simulink model "pendulum_pid"  (R2025b)
settings: Solver=ode45  StartTime=0.0  StopTime=8  MaxStep=1e-3  RelTol=1e-6
values from neighbouring files (symbols this model uses):
  A = reshape(p(1:16),4,4)    [main_pid_inverted_pendulum.m]    (also in params.m = [0  1         0                  0)
  B = p(17:20)'; [Kp,Ki,Kd,N] = deal(p(21),p(22),p(23),p(24))    [main_pid_inverted_pendulum.m]    (also in params.m = [0; J/D; 0; -m*l/D])
  Cfull = eye(4)    [compare_pid_vs_assy.m]
  Dfull = zeros(4,1)    [build_simulink_pid_model.m]    (also in compare_pid_vs_assy.m)
  Kd = -645.6    [main_pid_inverted_pendulum.m]    (also in optimize_pid.m = K(3); pid_gains.mat)
  Ki = -8365.6    [main_pid_inverted_pendulum.m]    (also in optimize_pid.m = K(2); pid_gains.mat)
  Kp = -4192.9    [main_pid_inverted_pendulum.m]    (also in optimize_pid.m = K(1); pid_gains.mat)
  Tf = 1/100    (= 0.01)    [main_pid_inverted_pendulum.m]    (also in optimize_pid.m; pid_gains.mat)
  th0 = asin(0.023848750116849705)    [params.m]
  x0 = [0; 0; th0; 0]    [build_simulink_pid_model.m]    (also in compare_pid_vs_assy.m; optimize_pid.m = [0;0;1;0;0;-1])
libraries: slpidlib x1
settings Model: Creator=kSam  LastModifiedBy=kSam

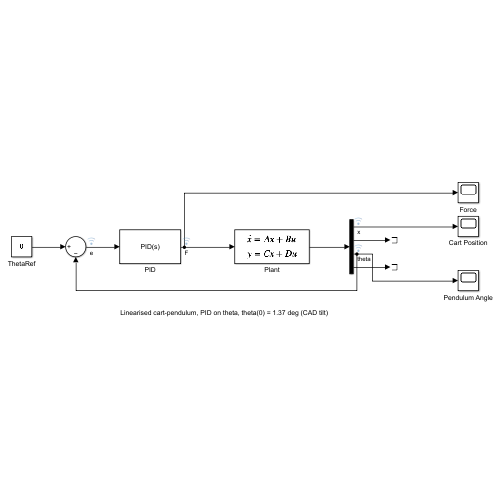
[thumbnail: Simulink's stored preview of the top-level diagram]
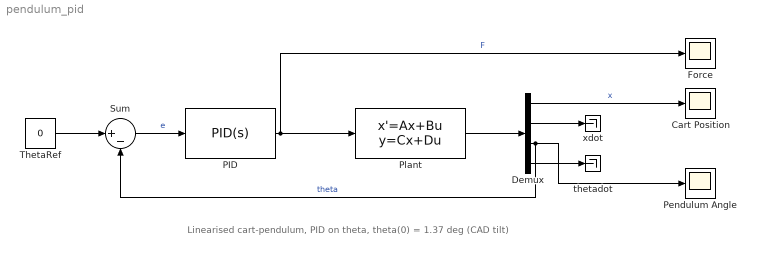
== system pendulum_pid ==
  note: Linearised cart-pendulum, PID on theta, theta(0) = 1.37 deg (CAD tilt)
  Cart Position : Scope
      settings: TimeSpan=8  Title=Cart position x  ActiveDisplayYMinimum=-0.005  ActiveDisplayYMaximum=0.035  YLabel=x [m]
  Demux : Demux
  Force : Scope
      settings: TimeSpan=8  Title=Control force F  ActiveDisplayYMinimum=-20  ActiveDisplayYMaximum=110  YLabel=F [N]
  PID : slpidlib/PID Controller  Controller=PID  Form=Parallel  TimeDomain=Continuous-time  UseExternalTs=off  SampleTime=-1  IntegratorMethod=Forward Euler  FilterMethod=Forward Euler  ControllerParametersSource=internal  P=Kp  I=Ki  UseKiTs=off  D=Kd  UseExternalDerivativeSource=off  N=1/Tf  UseFilter=on  TunerSelectOption=Transfer Function Based (PID Tuner App)  InitialConditionSource=internal  InitialConditionForIntegrator=0  InitialConditionForFilter=Kd*(-th0)  DifferentiatorICPrevScaledInput=0  ExternalReset=none  TrackingMode=off  Kt=1  LimitOutput=off  SatLimitsSource=internal  UpperSaturationLimit=inf  LowerSaturationLimit=-inf  LinearizeAsGain=on  AntiWindupMode=none  Kb=1  LimitIntegrator=off  UpperIntegratorSaturationLimit=inf  LowerIntegratorSaturationLimit=-inf  POutMin=[]  POutMax=[]  IOutMin=[]  IOutMax=[]  DOutMin=[]  DOutMax=[]  NOutMin=[]  NOutMax=[]  SumOutMin=[]  SumOutMax=[]  SaturationOutMin=[]  SaturationOutMax=[]  PParamMin=[]  PParamMax=[]  IParamMin=[]  IParamMax=[]  DParamMin=[]  DParamMax=[]  NParamMin=[]  NParamMax=[]  KbParamMin=[]  KbParamMax=[]  KtParamMin=[]  KtParamMax=[]  KbOutMin=[]  KbOutMax=[]  KtOutMin=[]  KtOutMax=[]  IntegratorOutMin=[]  IntegratorOutMax=[]  FilterOutMin=[]  FilterOutMax=[]  SumI1OutMin=[]  SumI1OutMax=[]  SumI2OutMin=[]  SumI2OutMax=[]  SumI3OutMin=[]  SumI3OutMax=[]  SumI4OutMin=[]  SumI4OutMax=[]  SumDOutMin=[]  SumDOutMax=[]  DifferentiatorOutMin=[]  DifferentiatorOutMax=[]  FilterDiffOutCoefMin=[]  FilterDiffOutCoefMax=[]  ReciprocalOutMin=[]  ReciprocalOutMax=[]  SumDenOutMin=[]  SumDenOutMax=[]  SumNumOutMin=[]  SumNumOutMax=[]  DivideOutMin=[]  DivideOutMax=[]  UdiffTsProdOutMin=[]  UdiffTsProdOutMax=[]  NTsProdOutMin=[]  NTsProdOutMax=[]  UintegralTsProdOutMin=[]  UintegralTsProdOutMax=[]  UngainTsProdOutMin=[]  UngainTsProdOutMax=[]  ClampingZeroOutDataTypeStr=Inherit: Inherit via back propagation  ClampingZeroOutMin=[]  ClampingZeroOutMax=[]  FilterDenConstantOutDataTypeStr=Inherit: Inherit via back propagation  FilterDenConstantOutMin=[]  FilterDenConstantOutMax=[]  PCopyOutDataTypeStr=Inherit: Inherit via back propagation  PCopyOutMin=[]  PCopyOutMax=[]  NCopyOutDataTypeStr=Inherit: Inherit via back propagation  NCopyOutMin=[]  NCopyOutMax=[]  IntegratorContinuousStateAttributes=''  IntegratorStateMustResolveToSignalObject=off  IntegratorRTWStateStorageClass=Auto  FilterContinuousStateAttributes=''  FilterStateMustResolveToSignalObject=off  FilterRTWStateStorageClass=Auto  ParallelPVariant=InternalParameters  IdealPVariant=Disabled  IVariant=InternalParameters  DVariant=InternalParameters  IntegratorVariant=Continuous  SatVariant=Disabled  AWVariant=Passthrough  PCopyVariant=Disabled  TRVariant=Disabled  FdbkBlocksVariant=Forward  IdealPFdbkVariant=Disabled  SatFdbkVariant=Disabled  DerivativeFilterVariant=ContFilter  NVariant=InternalParameters  NCopyVariant=Disabled  FilterICVariant=InternalICsFilter  IntegratorICVariant=InternalICs  ExternalResetVariant=Disabled  TRSumVariant=Passthrough  SumFdbkVariant=Disabled  SumVariant=Sum_PID  TsampFilterVariant=InternalTs  TsampNgainVariant=Passthrough  TsampIntegralVariant=Disabled_SignalSpec  ExternalSaturationOutDataTypeStr=Inherit: Same as second input  DerivativeSourceVariant=ErrorSignal  PreIntVariant=InternalPreInt
  Pendulum Angle : Scope
      settings: TimeSpan=8  Title=Pendulum angle \theta  ActiveDisplayYMinimum=-0.01  ActiveDisplayYMaximum=0.025  YLabel=\theta [rad]
  Plant : StateSpace  A=A  B=B  C=Cfull  D=Dfull  InitialCondition=x0
  Sum : Sum  Inputs=|+-
  ThetaRef : Constant  Value=0
  thetadot : Terminator
  xdot : Terminator
  wires:
  ThetaRef/1 -> Sum/1
  Sum/1 -> PID/1  "e"
  PID/1 -> Plant/1, Force/1  "F"
  Plant/1 -> Demux/1
  Demux/1 -> Cart Position/1  "x"
  Demux/2 -> xdot/1
  Demux/3 -> Pendulum Angle/1, Sum/2  "theta"
  Demux/4 -> thetadot/1
